simulink model "CRM_model"  (R2021b)
settings: Solver=FixedStepAuto  StartTime=0.0  StopTime=T  FixedStep=dt  RelTol=1e-3  AbsTol=1e-3
values from neighbouring files (symbols this model uses):
  f =     [20230919_data_fit.mat]    (also in chenRinconMoraModel_optimization.m = @(SOC,p)  p(1)*exp(p(2)*SOC) + p(3)*SOC.^3 + p(4)*SOC.^2 + p; chenRinconMoraModel_simulate.m = @(SOC,p)  p(1)*exp(p(2)*SOC) + p(3)*SOC.^3 + p(4)*SOC.^2 + p; chenRinconMoraModel_simulate_expdata.m = @(SOC,p)  p(1)*exp(p(2)*SOC) + p(3)*SOC.^3 + p(4)*SOC.^2 + p; test2_paramFit.m = @(SOC,p)  p(1)*exp(p(2)*SOC) + p(3)*SOC.^3 + p(4)*SOC.^2 + p)
  g =     [20230919_data_fit.mat]    (also in chenRinconMoraModel_optimization.m = @(SOC,p)  p(1).*exp(p(2).*SOC) + p(3); chenRinconMoraModel_simulate.m = @(SOC,p)  p(1).*exp(p(2).*SOC) + p(3); chenRinconMoraModel_simulate_expdata.m = @(SOC,p)  p(1).*exp(p(2).*SOC) + p(3); crm_paramfit.m = @(x,p)  p(1).*exp(p(2).*x) + p(3))
  p = zeros(size(yp,1),3)    [crm_paramfit.m]    (also in psObj_correction.m = Pulse(i))
  X_0 = 0.89    [chenRinconMoraModel_simulate_expdata.m]
  X_L = 0.013168 + 0.01646    (= 0.029628)    [chenRinconMoraModel_simulate_expdata.m]
  X_NA = 0.01    [chenRinconMoraModel_simulate_expdata.m]
libraries: fl_lib x14, nesl_utility x13, ee_lib x3, dspstat3 x2
settings Model: Creator=drkfr  LastModifiedBy=drkfr
settings SolverCC: AutoScaleAbsTol=off
settings DebuggingCC: SymbolicDimsDataTypeCodeGenerationDiagnostic=none  SFMachineParentedDataDiag=warning
settings SFSimCC: CustomCodeUndefinedFunction=UseInterfaceOnly
settings SimscapeCC: SimscapeLogType=all  SimscapeLogSimulationStatistics=on  SimscapeLogDataHistory=10000

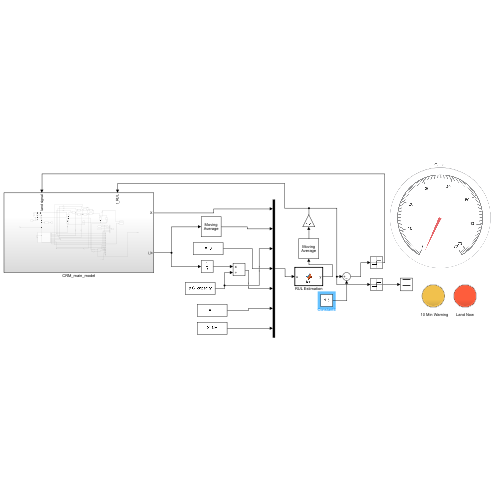
[thumbnail: Simulink's stored preview of the top-level diagram]
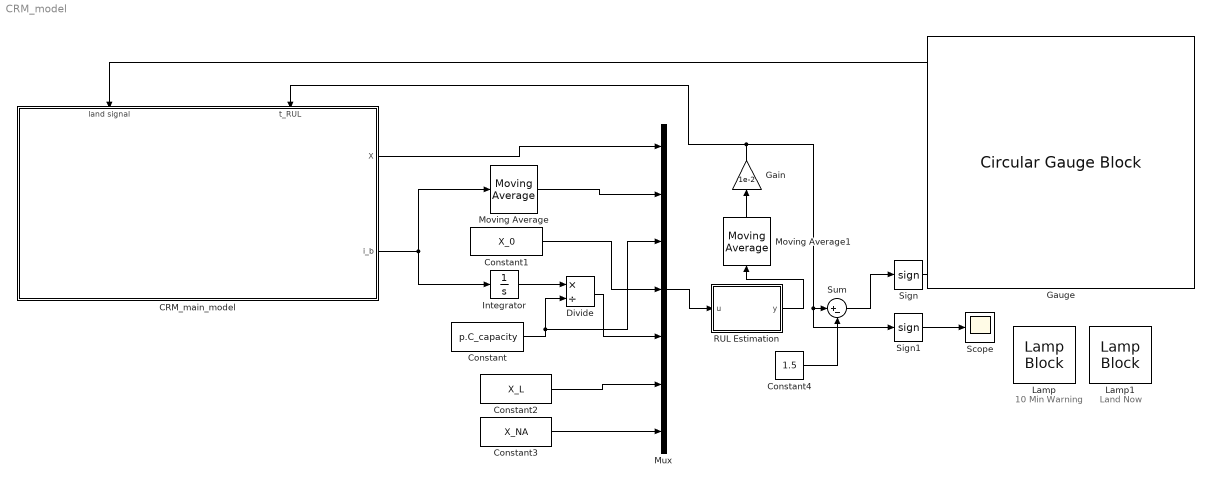
== system CRM_model ==
  note: 10 Min Warning
  note: Land Now
  CRM_main_model : Subsystem
      settings: PortSchema="{\"entries\":[{\"content\":{\"sides\":[{\"content\":{\"connectorIds\":[]},\"type\":\"ConnectorPlacement.EquallySpacedRectSide\",\"uuid\":\"7561b6b1-3e3a-4e84-a2eb-edcb3907bb51\"},{\"content\":{\"connectorIds\":[\"Out1\",\"Out2\"],\"side\":\"RIGHT\"},\"type\":\"ConnectorPlacement.EquallySpacedRectSide\",\"uuid\":\"041a36de-4d85-4d3d-b193-79c04204387c\"},{\"content\":{\"connectorIds\":[\"In1\",\"In2\"],\"side\":\"TOP\"},\"type\":\"ConnectorPlacement.EquallySpacedRectSide\",\"uuid\":\"4dc0730b-c175-4d57-a51c-0a7e8a18dfb4\"}]},\"type\":\"ConnectorPlacement.EquallySpacedConnector\",\"uuid\":\"326e57a0-6394-41a2-ac3f-5fdca9005cf7\"}],\"packageUris\":[\"http://schema.mathworks.com/mf0/Connector/R2020b\"],\"version\":\"1.0\"}"
  Constant : Constant  Value=p.C_capacity
  Constant1 : Constant  Value=X_0
  Constant2 : Constant  Value=X_L
  Constant3 : Constant  Value=X_NA
  Constant4 : Constant  Value=1.5
  Divide : Product  Inputs=*/
  Gain : Gain  Gain=1e-2
  Gauge : CircularGaugeBlock  ScaleMax=72  TickInterval=10
  Integrator : Integrator
  Lamp : LampBlock  LabelPosition=Hide
  Lamp1 : LampBlock  LabelPosition=Hide
  Moving Average : dspstat3/Moving Average  Method=Sliding window  ForgettingFactorPort=off  SpecifyWindowLength=on  WindowLength=1000  ForgettingFactor=0.9  SimulateUsing=Code generation
  Moving Average1 : dspstat3/Moving Average  Method=Sliding window  ForgettingFactorPort=off  SpecifyWindowLength=on  WindowLength=1000  ForgettingFactor=0.9  SimulateUsing=Code generation
  Mux : Mux  Inputs=7
  RUL Estimation : MATLAB Function  TreatAsAtomicUnit=on
  Scope : Scope
  Sign : Signum
  Sign1 : Signum
  Sum : Sum  Inputs=|+-
  wires:
  CRM_main_model/2(i_b) -> Integrator/1, Moving Average/1
  Constant/1 -> Mux/3, Divide/2
  Integrator/1 -> Divide/1
  Mux/1 -> RUL Estimation/1(u)
  CRM_main_model/1(X) -> Mux/1
  Moving Average/1 -> Mux/2
  Constant1/1 -> Mux/4
  Divide/1 -> Mux/5
  Constant2/1 -> Mux/6
  Constant3/1 -> Mux/7
  RUL Estimation/1(y) -> Moving Average1/1
  Moving Average1/1 -> Gain/1
  Gain/1 -> Sign1/1, Sum/1, CRM_main_model/2(t_RUL)
  Sum/1 -> Sign/1
  Constant4/1 -> Sum/2
  Sign/1 -> CRM_main_model/1(land signal)
  Sign1/1 -> Scope/1

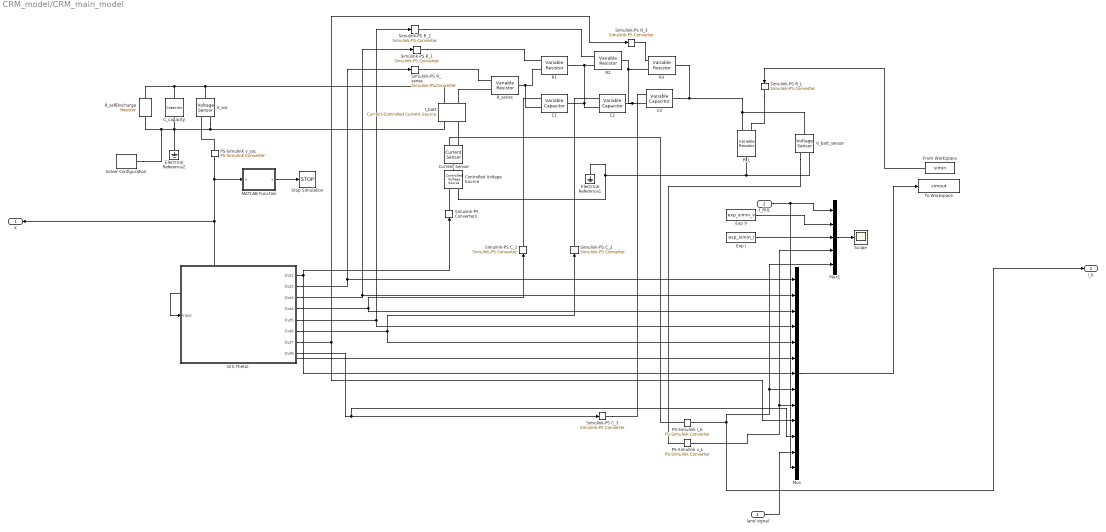
== system CRM_model/CRM_main_model ==
  land signal : Inport
  t_RUL : Inport  Port=2
  C1 : ee_lib/Passive/Variable Capacitor  prm=2  Cmin=1e-9 F  r=1e-6 Ohm  v0=0 V  q0=0 C
      settings: SourceProductBaseCode=PS  InternalSimscapePortConfiguration="{\"Bottom\":[],\"Left\":[{\"id\":\"C\",\"label\":\"C\",\"type\":\"input\"},{\"id\":\"p\",\"label\":\"+\",\"type\":\"foundation.electrical.electrical\"}],\"Right\":[{\"id\":\"n\",\"label\":\"-\",\"type\":\"foundation.electrical.electrical\"}],\"Top\":[]}"
  C2 : ee_lib/Passive/Variable Capacitor  prm=2  Cmin=1e-9 F  r=1e-6 Ohm  v0=0 V  q0=0 C
      settings: SourceProductBaseCode=PS  InternalSimscapePortConfiguration="{\"Bottom\":[],\"Left\":[{\"id\":\"C\",\"label\":\"C\",\"type\":\"input\"},{\"id\":\"p\",\"label\":\"+\",\"type\":\"foundation.electrical.electrical\"}],\"Right\":[{\"id\":\"n\",\"label\":\"-\",\"type\":\"foundation.electrical.electrical\"}],\"Top\":[]}"
  C3 : ee_lib/Passive/Variable Capacitor  prm=2  Cmin=1e-9 F  r=1e-6 Ohm  v0=0 V  q0=0 C
      settings: SourceProductBaseCode=PS  InternalSimscapePortConfiguration="{\"Bottom\":[],\"Left\":[{\"id\":\"C\",\"label\":\"C\",\"type\":\"input\"},{\"id\":\"p\",\"label\":\"+\",\"type\":\"foundation.electrical.electrical\"}],\"Right\":[{\"id\":\"n\",\"label\":\"-\",\"type\":\"foundation.electrical.electrical\"}],\"Top\":[]}"
  C_capacity : fl_lib/Electrical/Electrical Elements/Capacitor  c=p.C_capacity F  r=1e-6 Ohm  g=0 1/Ohm  i_specify=off  i_priority=None  i=0 A  i_nominal_specify=off  i_nominal_unit=A  i_nominal_value=1  v_specify=off  v_priority=None  v=50 V  v_nominal_specify=off  v_nominal_unit=V  v_nominal_value=1  vc_specify=on  vc_priority=High  vc=v.SOC V  vc_nominal_specify=off  vc_nominal_unit=V  vc_nominal_value=1
  Controlled Voltage Source : fl_lib/Electrical/Electrical Sources/Controlled Voltage Source
  Current Sensor : fl_lib/Electrical/Electrical Sensors/Current Sensor
  Electrical Reference1 : fl_lib/Electrical/Electrical Elements/Electrical Reference
  Electrical Reference2 : fl_lib/Electrical/Electrical Elements/Electrical Reference
  Exp I : FromWorkspace  VariableName=exp_simin_i
  Exp V : FromWorkspace  VariableName=exp_simin_v
  From Workspace : FromWorkspace  VariableName=simin
  G(X,Theta) : Subsystem
  I_batt : fl_lib/Electrical/Electrical Sources/Current-Controlled Current Source  K=1  i1_specify=off  i1_priority=None  i1=0 A  i1_nominal_specify=off  i1_nominal_unit=A  i1_nominal_value=1  i2_specify=off  i2_priority=None  i2=0 A  i2_nominal_specify=off  i2_nominal_unit=A  i2_nominal_value=1
      settings: SourceProductBaseCode=SS  InternalSimscapePortConfiguration="{\"Bottom\":[],\"Left\":[{\"id\":\"p1\",\"label\":\"+\",\"type\":\"foundation.electrical.electrical\"},{\"id\":\"head\",\"label\":\"\",\"type\":\"foundation.electrical.electrical\"}],\"Right\":[{\"id\":\"n1\",\"label\":\"-\",\"type\":\"foundation.electrical.electrical\"},{\"id\":\"tail\",\"label\":\"\",\"type\":\"foundation.electrical.electrical\"}],\"Top\":[]}"
  MATLAB Function : MATLAB Function  TreatAsAtomicUnit=on
  Mux : Mux  Inputs=13
  Mux1 : Mux  Inputs=5
  PS-Simulink i_b : nesl_utility/PS-Simulink Converter  PhysicalDomain=network_engine_domain  SubClassName=ps_output  LeftPortType=input  RightPortType=output  PseudoPeriodic=off  Frequencies=[]  Unit=A  AffineConversion=off
      settings: SourceProductBaseCode=PW,SS
  PS-Simulink v_L : nesl_utility/PS-Simulink Converter  PhysicalDomain=network_engine_domain  SubClassName=ps_output  LeftPortType=input  RightPortType=output  PseudoPeriodic=off  Frequencies=[]  Unit=V  AffineConversion=off
      settings: SourceProductBaseCode=PW,SS
  PS-Simulink v_soc : nesl_utility/PS-Simulink Converter  PhysicalDomain=network_engine_domain  SubClassName=ps_output  LeftPortType=input  RightPortType=output  PseudoPeriodic=off  Frequencies=[]  Unit=V  AffineConversion=off
      settings: SourceProductBaseCode=PW,SS
  R1 : fl_lib/Electrical/Electrical Elements/Variable Resistor  Rmin=0 Ohm  i_specify=off  i_priority=None  i=0 A  i_nominal_specify=off  i_nominal_unit=A  i_nominal_value=1  v_specify=off  v_priority=None  v=0 V  v_nominal_specify=off  v_nominal_unit=V  v_nominal_value=1
  R2 : fl_lib/Electrical/Electrical Elements/Variable Resistor  Rmin=0 Ohm  i_specify=off  i_priority=None  i=0 A  i_nominal_specify=off  i_nominal_unit=A  i_nominal_value=1  v_specify=off  v_priority=None  v=0 V  v_nominal_specify=off  v_nominal_unit=V  v_nominal_value=1
  R3 : fl_lib/Electrical/Electrical Elements/Variable Resistor  Rmin=0 Ohm  i_specify=off  i_priority=None  i=0 A  i_nominal_specify=off  i_nominal_unit=A  i_nominal_value=1  v_specify=off  v_priority=None  v=0 V  v_nominal_specify=off  v_nominal_unit=V  v_nominal_value=1
  R_L : fl_lib/Electrical/Electrical Elements/Variable Resistor  Rmin=0 Ohm  i_specify=off  i_priority=None  i=0 A  i_nominal_specify=off  i_nominal_unit=A  i_nominal_value=1  v_specify=off  v_priority=None  v=0 V  v_nominal_specify=off  v_nominal_unit=V  v_nominal_value=1
  R_selfDischarge : fl_lib/Electrical/Electrical Elements/Resistor  R=p.R_selfDischarge Ohm  i_specify=off  i_priority=None  i=0 A  i_nominal_specify=off  i_nominal_unit=A  i_nominal_value=1  v_specify=off  v_priority=None  v=0 V  v_nominal_specify=off  v_nominal_unit=V  v_nominal_value=1
  R_series : fl_lib/Electrical/Electrical Elements/Variable Resistor  Rmin=0 Ohm  i_specify=off  i_priority=None  i=0 A  i_nominal_specify=off  i_nominal_unit=A  i_nominal_value=1  v_specify=off  v_priority=None  v=0 V  v_nominal_specify=off  v_nominal_unit=V  v_nominal_value=1
  Scope : Scope
  Simulink-PS C_1 : nesl_utility/Simulink-PS Converter  PhysicalDomain=network_engine_domain  SubClassName=ps_input  LeftPortType=input  RightPortType=output  PseudoPeriodic=off  Frequencies=[]  NoiseDistribution=none  NoiseParameters=[]  Unit=F  AffineConversion=off  FilteringAndDerivatives=provide  SimscapeFilterOrder=1  InputFilterTimeConstant=0.001  UdotUserProvided=0
      settings: SourceProductBaseCode=PW,SS
  Simulink-PS C_2 : nesl_utility/Simulink-PS Converter  PhysicalDomain=network_engine_domain  SubClassName=ps_input  LeftPortType=input  RightPortType=output  PseudoPeriodic=off  Frequencies=[]  NoiseDistribution=none  NoiseParameters=[]  Unit=F  AffineConversion=off  FilteringAndDerivatives=provide  SimscapeFilterOrder=1  InputFilterTimeConstant=0.001  UdotUserProvided=0
      settings: SourceProductBaseCode=PW,SS
  Simulink-PS C_3 : nesl_utility/Simulink-PS Converter  PhysicalDomain=network_engine_domain  SubClassName=ps_input  LeftPortType=input  RightPortType=output  PseudoPeriodic=off  Frequencies=[]  NoiseDistribution=none  NoiseParameters=[]  Unit=F  AffineConversion=off  FilteringAndDerivatives=provide  SimscapeFilterOrder=1  InputFilterTimeConstant=0.001  UdotUserProvided=0
      settings: SourceProductBaseCode=PW,SS
  Simulink-PS Converter2 : nesl_utility/Simulink-PS Converter  PhysicalDomain=network_engine_domain  SubClassName=ps_input  LeftPortType=input  RightPortType=output  PseudoPeriodic=off  Frequencies=[]  NoiseDistribution=none  NoiseParameters=[]  Unit=V  AffineConversion=off  FilteringAndDerivatives=provide  SimscapeFilterOrder=1  InputFilterTimeConstant=0.001  UdotUserProvided=0
      settings: SourceProductBaseCode=PW,SS
  Simulink-PS R_1 : nesl_utility/Simulink-PS Converter  PhysicalDomain=network_engine_domain  SubClassName=ps_input  LeftPortType=input  RightPortType=output  PseudoPeriodic=off  Frequencies=[]  NoiseDistribution=none  NoiseParameters=[]  Unit=Ohm  AffineConversion=off  FilteringAndDerivatives=provide  SimscapeFilterOrder=1  InputFilterTimeConstant=0.001  UdotUserProvided=0
      settings: SourceProductBaseCode=PW,SS
  Simulink-PS R_2 : nesl_utility/Simulink-PS Converter  PhysicalDomain=network_engine_domain  SubClassName=ps_input  LeftPortType=input  RightPortType=output  PseudoPeriodic=off  Frequencies=[]  NoiseDistribution=none  NoiseParameters=[]  Unit=Ohm  AffineConversion=off  FilteringAndDerivatives=provide  SimscapeFilterOrder=1  InputFilterTimeConstant=0.001  UdotUserProvided=0
      settings: SourceProductBaseCode=PW,SS
  Simulink-PS R_3 : nesl_utility/Simulink-PS Converter  PhysicalDomain=network_engine_domain  SubClassName=ps_input  LeftPortType=input  RightPortType=output  PseudoPeriodic=off  Frequencies=[]  NoiseDistribution=none  NoiseParameters=[]  Unit=Ohm  AffineConversion=off  FilteringAndDerivatives=provide  SimscapeFilterOrder=1  InputFilterTimeConstant=0.001  UdotUserProvided=0
      settings: SourceProductBaseCode=PW,SS
  Simulink-PS R_L : nesl_utility/Simulink-PS Converter  PhysicalDomain=network_engine_domain  SubClassName=ps_input  LeftPortType=input  RightPortType=output  PseudoPeriodic=off  Frequencies=[]  NoiseDistribution=none  NoiseParameters=[]  Unit=Ohm  AffineConversion=off  FilteringAndDerivatives=provide  SimscapeFilterOrder=1  InputFilterTimeConstant=0.001  UdotUserProvided=0
      settings: SourceProductBaseCode=PW,SS
  Simulink-PS R_series : nesl_utility/Simulink-PS Converter  PhysicalDomain=network_engine_domain  SubClassName=ps_input  LeftPortType=input  RightPortType=output  PseudoPeriodic=off  Frequencies=[]  NoiseDistribution=none  NoiseParameters=[]  Unit=Ohm  AffineConversion=off  FilteringAndDerivatives=provide  SimscapeFilterOrder=1  InputFilterTimeConstant=0.001  UdotUserProvided=0
      settings: SourceProductBaseCode=PW,SS
  Solver Configuration : nesl_utility/Solver Configuration  PhysicalDomain=network_engine_domain  SubClassName=solver  LeftPortType=input  RightPortType=generic  Tones=[]  Harmonics=[]  SimulateNoise=off  Profile=off  UseLocalSampling=off  EnableSwitchedLinearOptims=on  FrequencyDomain=off  UseCCode=off  RelTol=0.001  AbsTol=1e-06  MinStep=1e-09  ToWorkspace=off  RevertToSquareIcSolve=off  NumHomotopyIterations=100  PhasorMode=off  PhasorModeNumHarmonics=1  DoDC=on  ResidualTolerance=1e-09  UseLocalSolver=off  LocalSolverChoice=NE_BACKWARD_EULER_ADVANCER  LocalSolverSampleTime=0.001  DoFixedCost=off  MaxNonlinIter=3  MaxModeIter=2  ComputeImpulses=off  ImpulseIterations=2  LinearAlgebra=auto  EquationFormulation=NE_TIME_EF  DelaysMemoryBudget=1024  AutomaticFiltering=on  FilteringTimeConstant=0.001  PartitionStorageMethod=AS_NEEDED  PartitionMemoryBudget=1024  PartitionMethod=ROBUST
      settings: SourceProductBaseCode=PW,SS
  Stop Simulation : Stop
  To Workspace : ToWorkspace  VariableName=simout  SaveFormat=Timeseries  SampleTime=-1
  V_batt_sensor : fl_lib/Electrical/Electrical Sensors/Voltage Sensor
  V_soc : fl_lib/Electrical/Electrical Sensors/Voltage Sensor
  X : Outport
  i_b : Outport  Port=2
  wires:
  PS-Simulink v_soc/1 -> MATLAB Function/1(u), X/1, Mux/6, G(X,Theta)/1(Input)
  PS-Simulink i_b/1 -> i_b/1, Mux1/5, Mux/8
  MATLAB Function/1(y) -> Stop Simulation/1
  G(X,Theta)/3(Out3) -> Simulink-PS R_1/1, Mux/2
  G(X,Theta)/1(Out1) -> Simulink-PS Converter2/1, Mux/7
  PS-Simulink v_L/1 -> Mux1/4, Mux/9
  G(X,Theta)/4(Out4) -> Mux/3, Simulink-PS C_1/1
  G(X,Theta)/2(Out2) -> Simulink-PS R_series/1, Mux/1
  G(X,Theta)/7(Out7) -> Mux/10, Simulink-PS R_3/1
  Mux1/1 -> Scope/1
  From Workspace/1 -> Simulink-PS R_L/1
  G(X,Theta)/8(Out8) -> Mux/11, Simulink-PS C_3/1
  G(X,Theta)/5(Out5) -> Mux/4, Simulink-PS R_2/1
  Exp V/1 -> Mux1/2
  Exp I/1 -> Mux1/3
  Mux/1 -> To Workspace/1
  G(X,Theta)/6(Out6) -> Mux/5, Simulink-PS C_2/1
  t_RUL/1 -> Mux/13, Mux1/1
  land signal/1 -> Mux/12
  connections:
  I_batt/LConn2 -- R_selfDischarge/RConn1 -- Solver Configuration/RConn1 -- C_capacity/RConn1 -- Electrical Reference2/LConn1 -- V_soc/RConn2
  R1/RConn1 -- R2/LConn2 -- C2/LConn2 -- C1/RConn1
  R_series/RConn1 -- C1/LConn2 -- R1/LConn2
  Simulink-PS R_series/RConn1 -- R_series/LConn1
  C2/RConn1 -- R3/LConn2 -- R2/RConn1 -- C3/LConn2
  PS-Simulink i_b/LConn1 -- Current Sensor/RConn1
  Controlled Voltage Source/RConn2 -- Electrical Reference1/LConn1 -- R_L/RConn1 -- V_batt_sensor/RConn2
  Simulink-PS R_2/RConn1 -- R2/LConn1
  C_capacity/LConn1 -- V_soc/LConn1 -- I_batt/RConn2 -- R_selfDischarge/LConn1
  Current Sensor/LConn1 -- Controlled Voltage Source/LConn1
  Simulink-PS R_3/RConn1 -- R3/LConn1
  R_series/LConn2 -- I_batt/RConn1
  Simulink-PS C_1/RConn1 -- C1/LConn1
  Simulink-PS R_1/RConn1 -- R1/LConn1
  Simulink-PS C_2/RConn1 -- C2/LConn1
  R_L/LConn2 -- R3/RConn1 -- C3/RConn1 -- V_batt_sensor/LConn1
  Current Sensor/RConn2 -- I_batt/LConn1
  Simulink-PS C_3/RConn1 -- C3/LConn1
  V_batt_sensor/RConn1 -- PS-Simulink v_L/LConn1
  Controlled Voltage Source/RConn1 -- Simulink-PS Converter2/RConn1
  Simulink-PS R_L/RConn1 -- R_L/LConn1
  PS-Simulink v_soc/LConn1 -- V_soc/RConn1

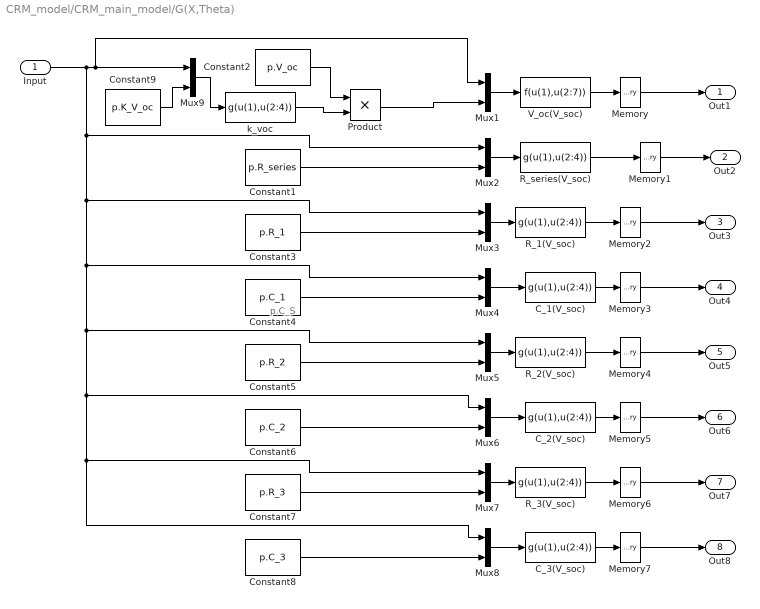
== system CRM_model/CRM_main_model/G(X,Theta) ==
  note: p.C_S
  Input : Inport
  C_1(V_soc) : MATLABFcn  MATLABFcn=g(u(1),u(2:4))  OutputDimensions=1
  C_2(V_soc) : MATLABFcn  MATLABFcn=g(u(1),u(2:4))  OutputDimensions=1  OutputSignalType=real
  C_3(V_soc) : MATLABFcn  MATLABFcn=g(u(1),u(2:4))  OutputDimensions=1  OutputSignalType=real
  Constant1 : Constant  Value=p.R_series
  Constant2 : Constant  Value=p.V_oc
  Constant3 : Constant  Value=p.R_1
  Constant4 : Constant  Value=p.C_1
  Constant5 : Constant  Value=p.R_2
  Constant6 : Constant  Value=p.C_2
  Constant7 : Constant  Value=p.R_3
  Constant8 : Constant  Value=p.C_3
  Constant9 : Constant  Value=p.K_V_oc
  Memory{,1..7} (8 alike) : Memory
  Mux{1..9} (9 alike) : Mux  Inputs=2
  Product : Product
  R_1(V_soc) : MATLABFcn  MATLABFcn=g(u(1),u(2:4))  OutputDimensions=1  OutputSignalType=real
  R_2(V_soc) : MATLABFcn  MATLABFcn=g(u(1),u(2:4))  OutputDimensions=1  OutputSignalType=real
  R_3(V_soc) : MATLABFcn  MATLABFcn=g(u(1),u(2:4))  OutputDimensions=1  OutputSignalType=real
  R_series(V_soc) : MATLABFcn  MATLABFcn=g(u(1),u(2:4))  OutputDimensions=1  OutputSignalType=real
  V_oc(V_soc) : MATLABFcn  MATLABFcn=f(u(1),u(2:7))  OutputDimensions=1  OutputSignalType=real
  k_voc : MATLABFcn  MATLABFcn=g(u(1),u(2:4))  OutputDimensions=1  OutputSignalType=real  Output1D=off
  Out1 : Outport
  Out2 : Outport  Port=2
  Out3 : Outport  Port=3
  Out4 : Outport  Port=4
  Out5 : Outport  Port=5
  Out6 : Outport  Port=6
  Out7 : Outport  Port=7
  Out8 : Outport  Port=8
  wires:
  V_oc(V_soc)/1 -> Memory/1
  Mux1/1 -> V_oc(V_soc)/1
  Memory/1 -> Out1/1
  Mux2/1 -> R_series(V_soc)/1
  R_series(V_soc)/1 -> Memory1/1
  Constant1/1 -> Mux2/2
  Mux3/1 -> R_1(V_soc)/1
  R_1(V_soc)/1 -> Memory2/1
  Constant3/1 -> Mux3/2
  Mux4/1 -> C_1(V_soc)/1
  C_1(V_soc)/1 -> Memory3/1
  Constant4/1 -> Mux4/2
  Constant6/1 -> Mux6/2
  C_2(V_soc)/1 -> Memory5/1
  Mux6/1 -> C_2(V_soc)/1
  R_2(V_soc)/1 -> Memory4/1
  Constant5/1 -> Mux5/2
  Mux5/1 -> R_2(V_soc)/1
  Memory1/1 -> Out2/1
  Memory5/1 -> Out6/1
  Memory4/1 -> Out5/1
  Memory3/1 -> Out4/1
  Memory2/1 -> Out3/1
  Mux8/1 -> C_3(V_soc)/1
  Constant8/1 -> Mux8/2
  Constant7/1 -> Mux7/2
  Mux7/1 -> R_3(V_soc)/1
  R_3(V_soc)/1 -> Memory6/1
  C_3(V_soc)/1 -> Memory7/1
  Memory7/1 -> Out8/1
  Input/1 -> Mux9/1, Mux1/1, Mux8/1, Mux7/1, Mux6/1, Mux5/1, Mux4/1, Mux3/1, Mux2/1
  Memory6/1 -> Out7/1
  Constant9/1 -> Mux9/2
  Mux9/1 -> k_voc/1
  k_voc/1 -> Product/2
  Constant2/1 -> Product/1
  Product/1 -> Mux1/2

== matlab function CRM_model/CRM_main_model/MATLAB Function ==
  data: u input; y output
function y = fcn(u)
if u <= 0
    y = 1;
else
    y = 0;
end

== matlab function CRM_model/RUL Estimation ==
  data: u input; y output
function y = fcn(u)
X = u(1);
ibar = u(2);
C = u(3);
X_0 = u(4);
X_i = u(5);
X_L = u(6);
X_NA = u(7);

X_RUL = X_0 - X_i - X_L - X_NA;
t_RUL = C*X_RUL/ibar;
y = t_RUL;
